simulink subsystem "ifft2d"  (R2024b)
settings: Solver=VariableStepAuto  StartTime=0.0  StopTime=10.0  RelTol=1e-3
undefined symbols (not defined in the file): B, K, L, LOG2L, NKEEP
libraries: hdlsllib x19, dsphdlxfrm2 x1
settings Model: Creator=User  LastModifiedBy=User

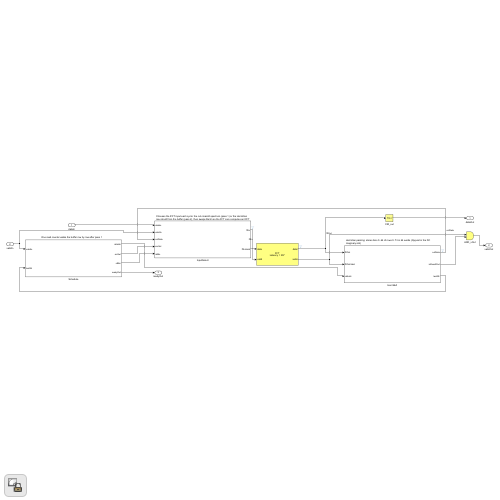
[thumbnail: Simulink's stored preview of the top-level diagram]
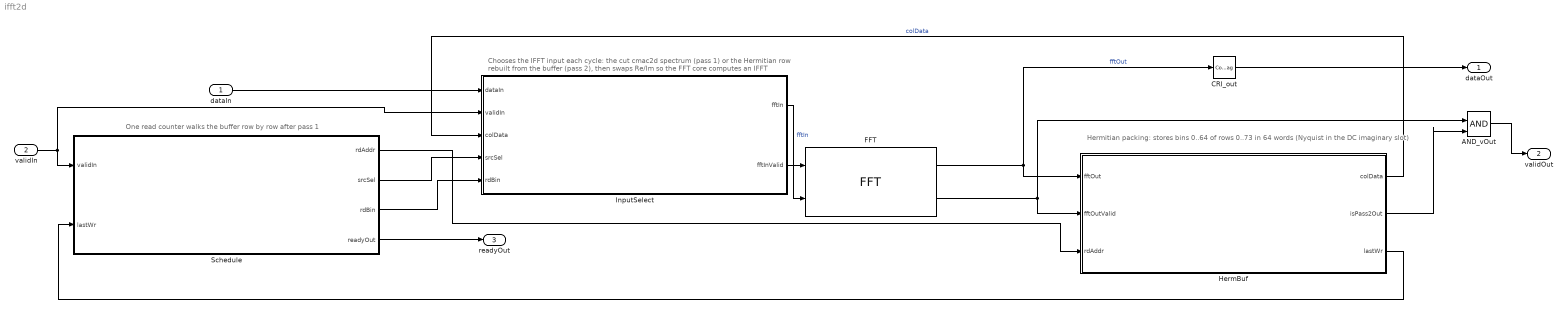
== system ifft2d ==
  note: Hermitian packing: stores bins 0..64 of rows 0..73 in 64 words (Nyquist in the DC imaginary slot)
  note: Chooses the IFFT input each cycle: the cut cmac2d spectrum (pass 1) or the Hermitian row rebuilt from the buffer (pass 2), then swaps Re/Im so the FFT core computes an IFFT
  note: One read counter walks the buffer row by row after pass 1
  dataIn : Inport  OutDataTypeStr=fixdt(1,ACC_WL,0)
      settings: SignalType=complex
  validIn : Inport  Port=2
  AND_vOut : Logic  IconShape=distinctive  AllPortsSameDT=off  OutDataTypeStr=boolean
  CRI_out : ComplexToRealImag  Output=Imag
  FFT : dsphdlxfrm2/FFT  Architecture=Streaming Radix 2^2  FFTLengthSource=Property  FFTLength=L  FFTLengthMax=1024  ComplexMultiplication=Use 4 multipliers and 2 adders  BitReversedOutput=off  BitReversedInput=off  Normalize=off  SimulateUsing=Code generation  RoundingMethod=Nearest  ResetInputPort=off  StartOutputPort=off  EndOutputPort=off
  HermBuf : Subsystem
  InputSelect : Subsystem
  Schedule : Subsystem
  dataOut : Outport  OutDataTypeStr=fixdt(1,IF_WL+LOG2L,0)
  validOut : Outport  Port=2
  readyOut : Outport  Port=3
  wires:
  Schedule/2(srcSel) -> InputSelect/4(srcSel)
  HermBuf/3(lastWr) -> Schedule/2(lastWr)
  validIn/1 -> Schedule/1(validIn), InputSelect/2(validIn)
  InputSelect/1(fftIn) -> FFT/1  "fftIn"
  Schedule/1(rdAddr) -> HermBuf/3(rdAddr)
  dataIn/1 -> InputSelect/1(dataIn)
  Schedule/3(rdBin) -> InputSelect/5(rdBin)
  Schedule/4(readyOut) -> readyOut/1
  InputSelect/2(fftInValid) -> FFT/2
  FFT/1 -> HermBuf/1(fftOut), CRI_out/1  "fftOut"
  FFT/2 -> HermBuf/2(fftOutValid), AND_vOut/1
  CRI_out/1 -> dataOut/1
  HermBuf/1(colData) -> InputSelect/3(colData)  "colData"
  HermBuf/2(isPass2Out) -> AND_vOut/2
  AND_vOut/1 -> validOut/1

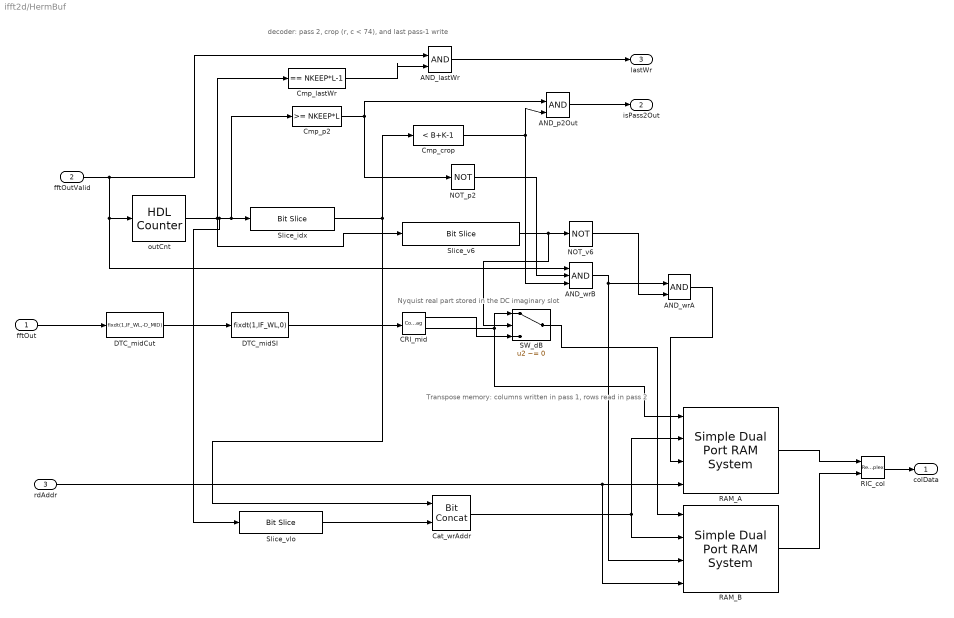
== system ifft2d/HermBuf ==
  note: Nyquist real part stored in the DC
      |  imaginary slot
  note: Transpose memory: columns written in pass 1, rows read in pass 2
  note: decoder: pass 2, crop (r, c < 74), and last pass-1 write
  fftOut : Inport  OutDataTypeStr=fixdt(1,IF_WL+LOG2L,0)
      settings: SignalType=complex
  fftOutValid : Inport  Port=2
  rdAddr : Inport  Port=3  OutDataTypeStr=fixdt(0,ceil(log2(B+K-1))+LOG2L-1,0)
  AND_lastWr : Logic  IconShape=distinctive  AllPortsSameDT=off  OutDataTypeStr=boolean
  AND_p2Out : Logic  IconShape=distinctive  AllPortsSameDT=off  OutDataTypeStr=boolean
  AND_wrA : Logic  IconShape=distinctive  AllPortsSameDT=off  OutDataTypeStr=boolean
  AND_wrB : Logic  Inputs=3  IconShape=distinctive  AllPortsSameDT=off  OutDataTypeStr=boolean
  CRI_mid : ComplexToRealImag
  Cat_wrAddr : hdlsllib/Logic and Bit Operations/Bit Concat  numInputs=2
  Cmp_crop : hdlsllib/Logic and Bit Operations/Compare To Constant  relop=<  const=B+K-1  OutDataTypeStr=boolean
  Cmp_lastWr : hdlsllib/Logic and Bit Operations/Compare To Constant  relop===  const=NKEEP*L-1  OutDataTypeStr=boolean
  Cmp_p2 : hdlsllib/Logic and Bit Operations/Compare To Constant  relop=>=  const=NKEEP*L  OutDataTypeStr=boolean
  DTC_midCut : DataTypeConversion  OutDataTypeStr=fixdt(1,IF_WL,-D_MID)  RndMeth=Nearest  SaturateOnIntegerOverflow=off
  DTC_midSI : DataTypeConversion  OutDataTypeStr=fixdt(1,IF_WL,0)  ConvertRealWorld=Stored Integer (SI)  SaturateOnIntegerOverflow=off  RndMeth=Floor
  NOT_p2 : Logic  Operator=NOT  IconShape=distinctive  AllPortsSameDT=off  OutDataTypeStr=boolean
  NOT_v6 : Logic  Operator=NOT  IconShape=distinctive  AllPortsSameDT=off  OutDataTypeStr=boolean
  RAM_A : hdlsllib/HDL RAMs/Simple Dual Port RAM System  RAMType=Simple dual port  AsyncRead=off  WriteOutputValue=New data  RAMInitialValue=0  allowBusInputs=off  WritesHaveOutput=on  NumReads=0  NumWrites=1  SimulateUsing=Code generation  ModelRAMDelay=on
  RAM_B : hdlsllib/HDL RAMs/Simple Dual Port RAM System  RAMType=Simple dual port  AsyncRead=off  WriteOutputValue=New data  RAMInitialValue=0  allowBusInputs=off  WritesHaveOutput=on  NumReads=0  NumWrites=1  SimulateUsing=Code generation  ModelRAMDelay=on
  RIC_col : RealImagToComplex
  SW_dB : Switch  Criteria=u2 ~= 0  OutDataTypeStr=fixdt(1,IF_WL,0)  SaturateOnIntegerOverflow=off  InputSameDT=off
  Slice_idx : hdlsllib/Logic and Bit Operations/Bit Slice  lidx=LOG2L-1  ridx=0
  Slice_v6 : hdlsllib/Logic and Bit Operations/Bit Slice  lidx=2*LOG2L-1  ridx=2*LOG2L-1
  Slice_vlo : hdlsllib/Logic and Bit Operations/Bit Slice  lidx=2*LOG2L-2  ridx=LOG2L
  outCnt : hdlsllib/Sources/HDL Counter  CountType=Count limited  CountInit=0  CountStep=1  CountMax=(NKEEP+B+K-1)*L-1  CountFromType=Initial value  CountFrom=0  CountResetPort=off  CountLoadPort=off  CountEnbPort=on  CountDirPort=off  CountHitOutputPort=off  CountDataType=Unsigned  CountWordLen=ceil(log2((NKEEP+B+K-1)*L))  CountFracLen=0  CountSampTime=1
  colData : Outport  OutDataTypeStr=fixdt(1,IF_WL,0)
      settings: SignalType=complex
  isPass2Out : Outport  Port=2
  lastWr : Outport  Port=3
  wires:
  RIC_col/1 -> colData/1
  RAM_B/1 -> RIC_col/2
  rdAddr/1 -> RAM_B/4, RAM_A/4
  RAM_A/1 -> RIC_col/1
  SW_dB/1 -> RAM_B/1
  NOT_v6/1 -> AND_wrA/2
  AND_p2Out/1 -> isPass2Out/1
  Cat_wrAddr/1 -> RAM_B/2, RAM_A/2
  CRI_mid/2 -> RAM_A/1, SW_dB/1
  Slice_v6/1 -> NOT_v6/1, SW_dB/2
  NOT_p2/1 -> AND_wrB/2
  Cmp_crop/1 -> AND_p2Out/2, AND_wrB/3
  Slice_vlo/1 -> Cat_wrAddr/2
  Slice_idx/1 -> Cat_wrAddr/1, Cmp_crop/1
  Cmp_lastWr/1 -> AND_lastWr/2
  DTC_midCut/1 -> DTC_midSI/1
  outCnt/1 -> Slice_v6/1, Cmp_lastWr/1, Slice_vlo/1, Slice_idx/1, Cmp_p2/1
  AND_lastWr/1 -> lastWr/1
  fftOut/1 -> DTC_midCut/1
  AND_wrB/1 -> AND_wrA/1, RAM_B/3
  AND_wrA/1 -> RAM_A/3
  Cmp_p2/1 -> AND_p2Out/1, NOT_p2/1
  DTC_midSI/1 -> CRI_mid/1
  CRI_mid/1 -> SW_dB/3
  fftOutValid/1 -> AND_lastWr/1, outCnt/1, AND_wrB/1

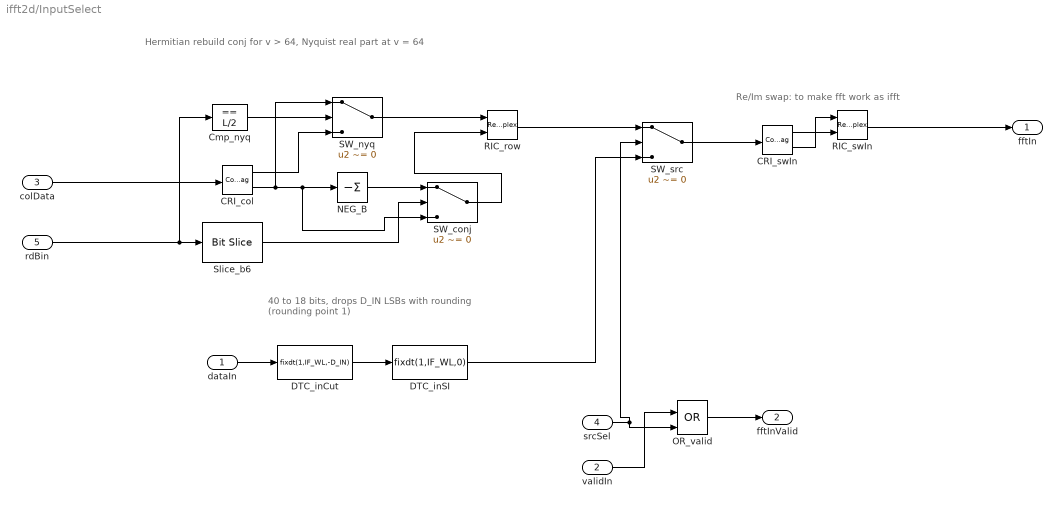
== system ifft2d/InputSelect ==
  note: Hermitian rebuild
      | conj for v > 64, Nyquist real part at v = 64
  note: Re/Im swap: to make fft work as ifft
  note: 40 to 18 bits, drops D_IN LSBs with
      | rounding (rounding point 1)
  dataIn : Inport  OutDataTypeStr=fixdt(1,ACC_WL,0)
      settings: SignalType=complex
  validIn : Inport  Port=2
  colData : Inport  Port=3  OutDataTypeStr=fixdt(1,IF_WL,0)
  srcSel : Inport  Port=4
  rdBin : Inport  Port=5  OutDataTypeStr=fixdt(0,LOG2L,0)
  CRI_col : ComplexToRealImag
  CRI_swIn : ComplexToRealImag
  Cmp_nyq : hdlsllib/Logic and Bit Operations/Compare To Constant  relop===  const=L/2  OutDataTypeStr=boolean
  DTC_inCut : DataTypeConversion  OutDataTypeStr=fixdt(1,IF_WL,-D_IN)  RndMeth=Nearest  SaturateOnIntegerOverflow=off
  DTC_inSI : DataTypeConversion  OutDataTypeStr=fixdt(1,IF_WL,0)  ConvertRealWorld=Stored Integer (SI)  RndMeth=Nearest  SaturateOnIntegerOverflow=off
  NEG_B : Sum  Inputs=-  OutDataTypeStr=fixdt(1,IF_WL,0)  AccumDataTypeStr=fixdt(1,IF_WL+1,0)
  OR_valid : Logic  Operator=OR  IconShape=distinctive  AllPortsSameDT=off  OutDataTypeStr=boolean
  RIC_row : RealImagToComplex
  RIC_swIn : RealImagToComplex
  SW_conj : Switch  Criteria=u2 ~= 0  OutDataTypeStr=fixdt(1,IF_WL,0)  SaturateOnIntegerOverflow=off  InputSameDT=off
  SW_nyq : Switch  Criteria=u2 ~= 0  OutDataTypeStr=fixdt(1,IF_WL,0)  SaturateOnIntegerOverflow=off  InputSameDT=off
  SW_src : Switch  Criteria=u2 ~= 0  OutDataTypeStr=fixdt(1,IF_WL,0)  SaturateOnIntegerOverflow=off  InputSameDT=off
  Slice_b6 : hdlsllib/Logic and Bit Operations/Bit Slice  lidx=LOG2L-1  ridx=LOG2L-1
  fftIn : Outport  OutDataTypeStr=fixdt(1,IF_WL,0)
      settings: SignalType=complex
  fftInValid : Outport  Port=2
  wires:
  RIC_swIn/1 -> fftIn/1
  CRI_swIn/1 -> RIC_swIn/2
  OR_valid/1 -> fftInValid/1
  SW_src/1 -> CRI_swIn/1
  validIn/1 -> OR_valid/1
  srcSel/1 -> OR_valid/2, SW_src/2
  DTC_inSI/1 -> SW_src/3
  DTC_inCut/1 -> DTC_inSI/1
  SW_conj/1 -> RIC_row/2
  dataIn/1 -> DTC_inCut/1
  Slice_b6/1 -> SW_conj/2
  CRI_col/2 -> SW_nyq/1, NEG_B/1, SW_conj/3
  RIC_row/1 -> SW_src/1
  NEG_B/1 -> SW_conj/1
  CRI_col/1 -> SW_nyq/3
  rdBin/1 -> Slice_b6/1, Cmp_nyq/1
  CRI_swIn/2 -> RIC_swIn/1
  Cmp_nyq/1 -> SW_nyq/2
  colData/1 -> CRI_col/1
  SW_nyq/1 -> RIC_row/1

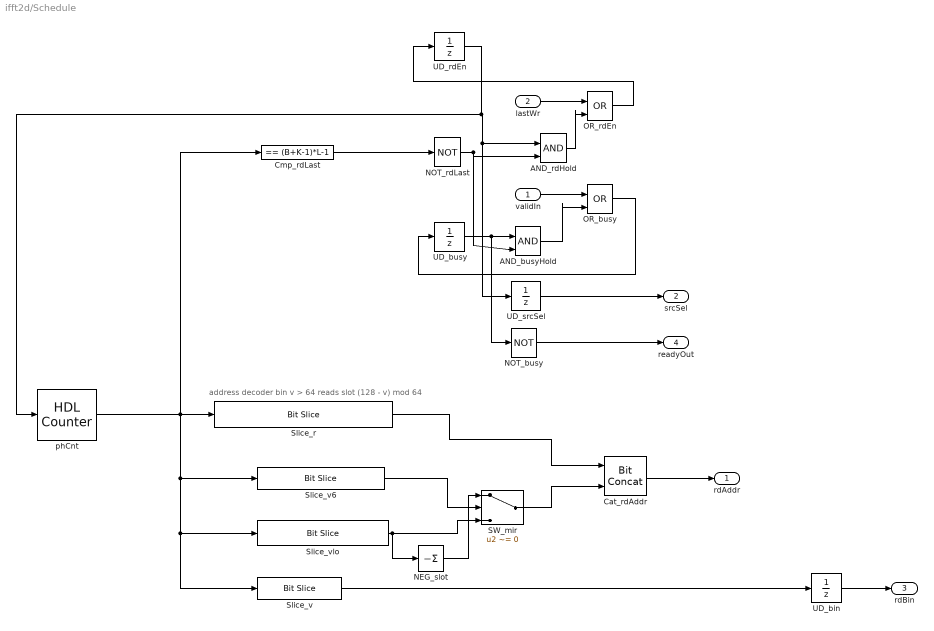
== system ifft2d/Schedule ==
  note: address decoder
      |
      |
      |
      |
      |
      |
      |
      |
      |
      |
      |
      |
      |
      |
      |
      |
      |
      |
      |
      | bin v > 64 reads slot (128 - v) mod 64
  validIn : Inport
  lastWr : Inport  Port=2
  AND_busyHold : Logic  IconShape=distinctive  AllPortsSameDT=off  OutDataTypeStr=boolean
  AND_rdHold : Logic  IconShape=distinctive  AllPortsSameDT=off  OutDataTypeStr=boolean
  Cat_rdAddr : hdlsllib/Logic and Bit Operations/Bit Concat  numInputs=2
  Cmp_rdLast : hdlsllib/Logic and Bit Operations/Compare To Constant  relop===  const=(B+K-1)*L-1  OutDataTypeStr=boolean
  NEG_slot : Sum  Inputs=-  OutDataTypeStr=fixdt(0,LOG2L-1,0)  AccumDataTypeStr=fixdt(1,LOG2L,0)
  NOT_busy : Logic  Operator=NOT  IconShape=distinctive  AllPortsSameDT=off  OutDataTypeStr=boolean
  NOT_rdLast : Logic  Operator=NOT  IconShape=distinctive  AllPortsSameDT=off  OutDataTypeStr=boolean
  OR_busy : Logic  Operator=OR  IconShape=distinctive  AllPortsSameDT=off  OutDataTypeStr=boolean
  OR_rdEn : Logic  Operator=OR  IconShape=distinctive  AllPortsSameDT=off  OutDataTypeStr=boolean
  SW_mir : Switch  Criteria=u2 ~= 0  OutDataTypeStr=fixdt(0,LOG2L-1,0)  SaturateOnIntegerOverflow=off  InputSameDT=off
  Slice_r : hdlsllib/Logic and Bit Operations/Bit Slice  lidx=ceil(log2(B+K-1))+LOG2L-1  ridx=LOG2L
  Slice_v : hdlsllib/Logic and Bit Operations/Bit Slice  lidx=LOG2L-1  ridx=0
  Slice_v6 : hdlsllib/Logic and Bit Operations/Bit Slice  lidx=LOG2L-1  ridx=LOG2L-1
  Slice_vlo : hdlsllib/Logic and Bit Operations/Bit Slice  lidx=LOG2L-2  ridx=0
  UD_bin : UnitDelay  SampleTime=-1  HasFrameUpgradeWarning=on
  UD_busy : UnitDelay  SampleTime=-1  HasFrameUpgradeWarning=on
  UD_rdEn : UnitDelay  SampleTime=-1  HasFrameUpgradeWarning=on
  UD_srcSel : UnitDelay  SampleTime=-1  HasFrameUpgradeWarning=on
  phCnt : hdlsllib/Sources/HDL Counter  CountType=Count limited  CountInit=0  CountStep=1  CountMax=(B+K-1)*L-1  CountFromType=Initial value  CountFrom=0  CountResetPort=off  CountLoadPort=off  CountEnbPort=on  CountDirPort=off  CountHitOutputPort=off  CountDataType=Unsigned  CountWordLen=ceil(log2(B+K-1))+LOG2L  CountFracLen=0  CountSampTime=1
  rdAddr : Outport
  srcSel : Outport  Port=2
  rdBin : Outport  Port=3
  readyOut : Outport  Port=4
  wires:
  Cat_rdAddr/1 -> rdAddr/1
  OR_busy/1 -> UD_busy/1
  OR_rdEn/1 -> UD_rdEn/1
  NOT_busy/1 -> readyOut/1
  UD_srcSel/1 -> srcSel/1
  AND_busyHold/1 -> OR_busy/2
  validIn/1 -> OR_busy/1
  lastWr/1 -> OR_rdEn/1
  UD_bin/1 -> rdBin/1
  NEG_slot/1 -> SW_mir/1
  UD_busy/1 -> AND_busyHold/1, NOT_busy/1
  Slice_v/1 -> UD_bin/1
  NOT_rdLast/1 -> AND_rdHold/2, AND_busyHold/2
  AND_rdHold/1 -> OR_rdEn/2
  SW_mir/1 -> Cat_rdAddr/2
  Slice_v6/1 -> SW_mir/2
  Slice_r/1 -> Cat_rdAddr/1
  Cmp_rdLast/1 -> NOT_rdLast/1
  UD_rdEn/1 -> AND_rdHold/1, UD_srcSel/1, phCnt/1
  phCnt/1 -> Cmp_rdLast/1, Slice_r/1, Slice_v6/1, Slice_vlo/1, Slice_v/1
  Slice_vlo/1 -> NEG_slot/1, SW_mir/3
